simulink subsystem "SimpleHydraulicPTO"  (R2025b)
settings: Solver=VariableStepAuto  StartTime=0.0  StopTime=10.0  RelTol=1e-3
libraries: customization_lib x4
settings Model: Creator=ndegoede  LastModifiedBy=ndegoede

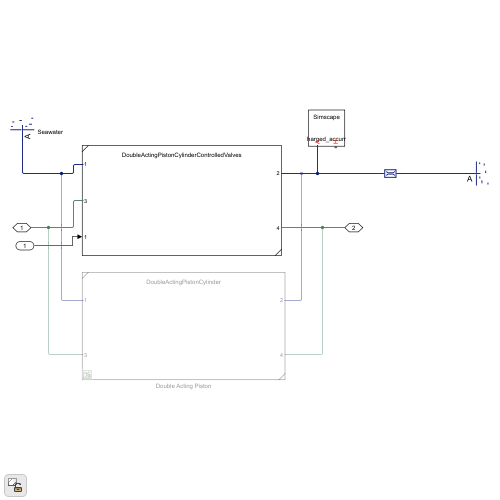
[thumbnail: Simulink's stored preview of the top-level diagram]
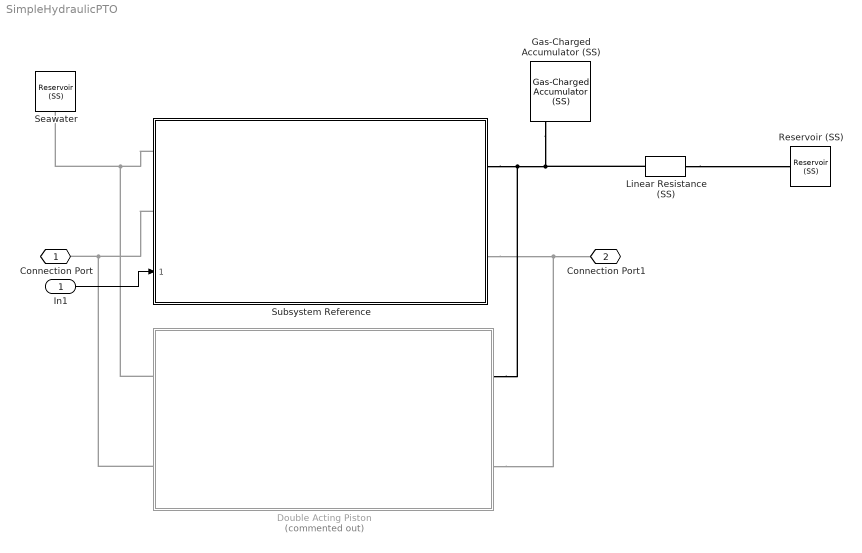
== system SimpleHydraulicPTO ==
  In1 : Inport
  " Seawater" : customization_lib/solution/elements/Reservoir (SS)  pressure_spec=foundation.enum.pressure_spec.specified  reservoir_pressure=P_ocean MPa  reservoir_temperature=293.15 K  reservoir_concentration=32 kg/m^3  area=0.1 m^2  custom_ports=false  length_A=1e-3 m
      settings: SourceProductName=Customization  InternalSimscapePortConfiguration="{\"Bottom\":[],\"Left\":[{\"id\":\"A\",\"label\":\"A\",\"type\":\"customization.solution.solution\"}],\"Right\":[],\"Top\":[]}"
  Double Acting Piston : Subsystem  Commented=on  ReferencedSubsystem=DoubleActingPistonCylinder
      settings: PortSchema="{\"entries\":[{\"content\":{\"sides\":[{\"content\":{\"connectorIds\":[\"LConn1\",\"LConn3\"]},\"type\":\"ConnectorPlacement.EquallySpacedRectSide\",\"uuid\":\"8acd0945-963f-4ac9-9e22-6ebef24fa469\"},{\"content\":{\"connectorIds\":[\"LConn2\",\"LConn4\"],\"side\":\"RIGHT\"},\"type\":\"ConnectorPlacement.EquallySpacedRectSide\",\"uuid\":\"3b4a74cd-deb1-4dcf-bacc-c9108daeb4d0\"},{\"content\":{\"side\":\"TOP\"},\"type\":\"ConnectorPlacement.EquallySpacedRectSide\",\"uuid\":\"b26b8698-1eb6-4b70-b966-bc7275cbd4a0\"},{\"content\":{\"side\":\"BOTTOM\"},\"type\":\"ConnectorPlacement.EquallySpacedRectSide\",\"uuid\":\"df97d8fb-7bd4-42c8-81cb-d93f7329400b\"}]},\"type\":\"ConnectorPlacement.EquallySpacedConnector\",\"uuid\":\"8ea66071-78df-4809-a2e0-9adf4b1871fd\"}],\"packageUris\":[\"http://schema.mathworks.com/mf0/Connector/R2020b\"],\"version\":\"1.0\"}"
  Gas-Charged Accumulator (SS) : customization_lib/solution/elements/Gas-Charged Accumulator (SS)  capacity=4 m^3  dead_volume=4e-5 m^3  p_precharge_gauge=2 MPa  k_sh=1.4  area=0.1 m^2  stiff_coeff=1e4 MPa/m^3  damping_coeff=1e4 MPa*s/m^6  custom_ports=false  length_A=1e-3 m  liquid_volume_specify=off  liquid_volume_priority=High  liquid_volume=5e-3 m^3  liquid_volume_nominal_specify=off  liquid_volume_nominal_value=1  liquid_volume_nominal_unit=m^3  liquid_mass_specify=off  liquid_mass_priority=None  liquid_mass=5 kg  liquid_mass_nominal_specify=off  liquid_mass_nominal_value=1  liquid_mass_nominal_unit=kg  p_I_specify=off  p_I_priority=High  p_I=P_ocean MPa  p_I_nominal_specify=off  p_I_nominal_value=1  p_I_nominal_unit=MPa  T_I_specify=off  T_I_priority=High  T_I=293.15 K  T_I_nominal_specify=off  T_I_nominal_value=1  T_I_nominal_unit=K  x_I_specify=off  x_I_priority=High  x_I=32 kg/m^3  x_I_nominal_specify=off  x_I_nominal_value=1  x_I_nominal_unit=kg/m^3
      settings: SourceProductName=Customization  InternalSimscapePortConfiguration="{\"Bottom\":[],\"Left\":[],\"Right\":[{\"id\":\"A\",\"label\":\"A\",\"type\":\"customization.solution.solution\"},{\"id\":\"H\",\"label\":\"H\",\"type\":\"foundation.thermal.thermal\"}],\"Top\":[]}"
  Linear Resistance (SS) : customization_lib/solution/elements/Linear Resistance (SS)  R=64.23e6 Pa*s/m^3  area=0.1 m^2  custom_ports=false  length_A=1e-3 m  length_B=1e-3 m
      settings: SourceProductName=Customization  InternalSimscapePortConfiguration="{\"Bottom\":[],\"Left\":[{\"id\":\"A\",\"label\":\"A\",\"type\":\"customization.solution.solution\"}],\"Right\":[{\"id\":\"B\",\"label\":\"B\",\"type\":\"customization.solution.solution\"}],\"Top\":[]}"
  Reservoir (SS) : customization_lib/solution/elements/Reservoir (SS)  pressure_spec=foundation.enum.pressure_spec.specified  reservoir_pressure=3 MPa  reservoir_temperature=293.15 K  reservoir_concentration=32 kg/m^3  area=0.1 m^2  custom_ports=false  length_A=1e-3 m
      settings: SourceProductName=Customization  InternalSimscapePortConfiguration="{\"Bottom\":[],\"Left\":[{\"id\":\"A\",\"label\":\"A\",\"type\":\"customization.solution.solution\"}],\"Right\":[],\"Top\":[]}"
  Subsystem Reference : Subsystem  ReferencedSubsystem=DoubleActingPistonCylinderControlledValves
      settings: PortSchema="{\"entries\":[{\"content\":{\"sides\":[{\"content\":{\"connectorIds\":[\"LConn1\",\"LConn3\",\"In1\"]},\"type\":\"ConnectorPlacement.EquallySpacedRectSide\",\"uuid\":\"cc974c7e-a23b-4542-9401-d7e5f7e305f2\"},{\"content\":{\"connectorIds\":[\"LConn2\",\"LConn4\"],\"side\":\"RIGHT\"},\"type\":\"ConnectorPlacement.EquallySpacedRectSide\",\"uuid\":\"6f9f7d00-9fe5-4287-8da4-035402e141b7\"},{\"content\":{\"side\":\"TOP\"},\"type\":\"ConnectorPlacement.EquallySpacedRectSide\",\"uuid\":\"ddb26387-7e3f-4441-bf36-3a3446a61f31\"}]},\"type\":\"ConnectorPlacement.EquallySpacedConnector\",\"uuid\":\"b4b61b79-bc73-49f9-a7b6-37286c37978d\"}],\"packageUris\":[\"http://schema.mathworks.com/mf0/Connector/R2020b\"],\"version\":\"1.0\"}"
  Connection Port : PMIOPort  Side=Left
  Connection Port1 : PMIOPort  Port=2  Side=Left
  wires:
  In1/1 -> Subsystem Reference/1
  connections:
  Double Acting Piston/LConn3 -- Subsystem Reference/LConn3 -- Connection Port/RConn1
  Double Acting Piston/LConn1 -- Subsystem Reference/LConn1 -- " Seawater"/LConn1
  Double Acting Piston/LConn4 -- Connection Port1/RConn1 -- Subsystem Reference/LConn4
  Subsystem Reference/LConn2 -- Gas-Charged Accumulator (SS)/RConn1 -- Linear Resistance (SS)/LConn1 -- Double Acting Piston/LConn2
  Linear Resistance (SS)/RConn1 -- Reservoir (SS)/LConn1
